simulink model "SigmoidSlidingModeObserverTest"  (R2026b)
settings: Solver=FixedStepDiscrete  StopTime=sigmoidTestCfg.Duration  FixedStep=sigmoidCfg.Ts
PostLoadFcn:
  | addpath(fullfile(fileparts(get_param(bdroot,'FileName')),'..','build_process'));initialize_sigmoid_smo_test(bdroot);
model workspace (MAT data in the model file):
  pllCfg.Ts = 5e-05
  pllCfg.NaturalFrequency = 40
  pllCfg.Damping = 0.707
  pllCfg.Kp = 355.376960974
  pllCfg.Ki = 63165.468167
  pllCfg.Kaw = 502.654824574
  pllCfg.OmegaMax = 1500
  pllCfg.MinMagnitude = 1
  pllCfg.LockError = 0.12
  pllCfg.LockSamples = 100
  pllCfg.Theta0 = 0
  pllCfg.Omega0 = 0
  sigmoidCfg.Ts = 5e-05
  sigmoidCfg.Rs = 0.5
  sigmoidCfg.L = 0.001
  sigmoidCfg.Flux = 0.035
  sigmoidCfg.PolePairs = 4
  sigmoidCfg.SlidingGain = 60
  sigmoidCfg.Slope = 0.6
  sigmoidCfg.MinEmf = 1
  sigmoidCfg.MinOmega = 30
  sigmoidCfg.MaxOmega = 800
  sigmoidCfg.MaxResidual = 2
  sigmoidCfg.MaxVoltage = 200
  sigmoidCfg.MaxCurrent = 20
  sigmoidCfg.MaxEstimate = 40
  sigmoidCfg.A = 0.975309912028
  sigmoidCfg.B = 0.0493801759433
  sigmoidCfg.MaximumInjectionSlope = 18
  sigmoidCfg.LocalErrorPole = 0.0864667450483
  sigmoidCfg.Settings = [0.975309912028; 0.0493801759433; 60; 0.6; 200; 20; 40]
  sigmoidTestCfg.Duration = 0.3
  sigmoidTestCfg.Omega = 200
  sigmoidTestCfg.InitialTheta = 0.4
  sigmoidTestCfg.Iq = 2
  sigmoidTestCfg.WindowStart = 0.25
  sigmoidTestCfg.MaximumAngleError = 0.08
  sigmoidTestCfg.MaximumSpeedRms = 15
  sigmoidTestCfg.MinimumValidFraction = 0.95
  sigmoidTestCfg.Seed = 23
  testStim.time = [0 5e-05 0.0001 0.00015 0.0002 0.00025 0.0003 0.00035 0.0004 0.00045 0.0005 0.00055 ... (6001 elements, 6001x1)]
  testStim.signals.values = [-3.48377113607 -3.555722953 -3.6273192006 -3.6985527193 -3.76941638582 -3.83990311383 -3.91000585473 -3.97971759831 -4.04903137344 -4.11794024881 -4.18643733359 -4.25451577812 ... (54009 elements, 6001x9)]
  testStim.signals.dimensions = 9
libraries: SigmoidSlidingModeObserver x1
settings Model: Creator=24322  LastModifiedBy=24322

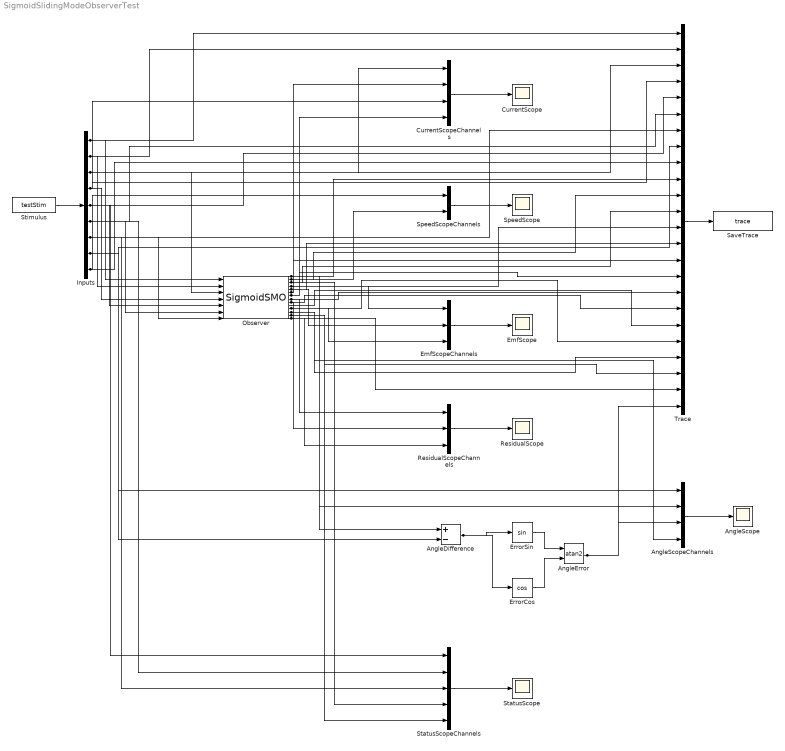
== system SigmoidSlidingModeObserverTest ==
  AngleDifference : Sum  Inputs=+-
  AngleError : Trigonometry  Operator=atan2
  AngleScope : Scope
  AngleScopeChannels : Mux
  CurrentScope : Scope
  CurrentScopeChannels : Mux
  EmfScope : Scope
  EmfScopeChannels : Mux  Inputs=3
  ErrorCos : Trigonometry  Operator=cos
  ErrorSin : Trigonometry
  Inputs : Demux  Outputs=9
  Observer : SigmoidSlidingModeObserver/SigmoidSMO  cfg=sigmoidCfg  trackerCfg=pllCfg
  ResidualScope : Scope
  ResidualScopeChannels : Mux  Inputs=3
  SaveTrace : ToWorkspace  VariableName=trace  SaveFormat=Structure With Time  SampleTime=sigmoidCfg.Ts
  SpeedScope : Scope
  SpeedScopeChannels : Mux  Inputs=2
  StatusScope : Scope
  StatusScopeChannels : Mux  Inputs=5
  Stimulus : FromWorkspace  VariableName=testStim  SampleTime=sigmoidCfg.Ts  Interpolate=off  OutputAfterFinalValue=Holding final value
  Trace : Mux  Inputs=24
  wires:
  StatusScopeChannels/1 -> StatusScope/1
  ResidualScopeChannels/1 -> ResidualScope/1
  CurrentScopeChannels/1 -> CurrentScope/1
  EmfScopeChannels/1 -> EmfScope/1
  SpeedScopeChannels/1 -> SpeedScope/1
  AngleScopeChannels/1 -> AngleScope/1
  Observer/14 -> Trace/23, ResidualScopeChannels/3
  Observer/13 -> Trace/22, StatusScopeChannels/5
  Observer/12 -> Trace/21, AngleScopeChannels/4
  Observer/11 -> Trace/20, EmfScopeChannels/3
  Observer/10 -> Trace/19
  Observer/9 -> Trace/18, ResidualScopeChannels/2
  Observer/8 -> Trace/17, ResidualScopeChannels/1
  Observer/7 -> Trace/16, CurrentScopeChannels/4
  Observer/6 -> Trace/15, CurrentScopeChannels/2
  Observer/5 -> Trace/14, EmfScopeChannels/2
  Observer/4 -> Trace/13, EmfScopeChannels/1
  Observer/3 -> Trace/12, StatusScopeChannels/4
  Observer/2 -> Trace/11, SpeedScopeChannels/2
  Inputs/9 -> Trace/9, SpeedScopeChannels/1
  Inputs/7 -> Observer/7, Trace/7, StatusScopeChannels/3
  Inputs/6 -> Trace/6, Observer/6, StatusScopeChannels/2
  Inputs/5 -> Trace/5, Observer/5, StatusScopeChannels/1
  Inputs/4 -> Observer/4, Trace/4, CurrentScopeChannels/3
  Inputs/3 -> Trace/3, Observer/3, CurrentScopeChannels/1
  Inputs/2 -> Trace/2, Observer/2
  Inputs/1 -> Trace/1, Observer/1
  AngleError/1 -> Trace/24, AngleScopeChannels/3
  ErrorCos/1 -> AngleError/2
  ErrorSin/1 -> AngleError/1
  AngleDifference/1 -> ErrorSin/1, ErrorCos/1
  Inputs/8 -> Trace/8, AngleDifference/2, AngleScopeChannels/1
  Observer/1 -> AngleDifference/1, Trace/10, AngleScopeChannels/2
  Trace/1 -> SaveTrace/1
  Stimulus/1 -> Inputs/1
